simulink library "half_bridge_three_level_ttype_mos_simple_2th"  (R2026a)
settings: Solver=VariableStepAuto
libraries: fl_lib x64, nesl_utility x40, mos_simple_2th_lib x4
(part 1 of 2)
settings Model: Creator=pwr-control  LastModifiedBy=pwr-control

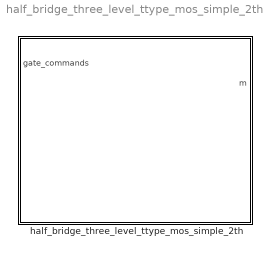
== system half_bridge_three_level_ttype_mos_simple_2th ==
  half_bridge_three_level_ttype_mos_simple_2th : Subsystem  mask(half_bridge_three_level_ttype_mos_simple_2th){rds_on_m=2.6, alpha_R_m=0, Tj_ref_m=125, Roff_m=1e7, v_gamma_m=4.5, rd_on_m=0.185, two_die_m=0, G_th_m=0.5, Eon_m=24, Eoff_m=8, Err_m=1.1, Ic_ref_m=450, Vdc_ref_m=600, ki_m=1, kv_m=1, Vth_off_m=50, Vth_on_m=25, V_sm_m=10, time_constant_edge_m=0.1, tau_v_m=10, time_constant_ploss_m=200, i_eps_m=1e-3, Csnubber_m=12e-12, Rsnubber_m=2200, rth_switch_JH_m=0.116, rth_switch_HA_m=0.05, rth_diode_JH_m=0.116, rth_diode_HA_m=0.05, JunctionTermalMass_m=0.2, Tambient_m=40, mass_heatsink_m=1, specific_heat_m=900}
      mask prompts: rds_on_m "On-state resistance at Tj_ref [mOhm]"; alpha_R_m "Rds_on temperature coefficient, 0 disables it [1/K]"; Tj_ref_m "Reference junction temperature of Rds_on [degC]"; Roff_m "Off-state resistance [Ohm]"; v_gamma_m "Diode knee voltage [V]"; rd_on_m "Diode differential resistance [mOhm]"; two_die_m "Diode die: 1 = separate die (losses to Hd), 0 = body diode (losses to Ht)"; G_th_m "Gate threshold: on when the gate command is above G_th"; Eon_m "Turn-on energy at Ic_ref, Vdc_ref [mJ]"; Eoff_m "Turn-off energy at Ic_ref, Vdc_ref [mJ]"; Err_m "Diode recovery energy at Ic_ref, Vdc_ref [mJ]"; Ic_ref_m "Reference current of the energies [A]"; Vdc_ref_m "Reference voltage of the energies [V]"; ki_m "Current exponent of the energy scaling"; kv_m "Voltage exponent of the energy scaling"; Vth_off_m "Turn-off / recovery detection threshold [V]"; Vth_on_m "Turn-on detection threshold (< Vth_off) [V]"; V_sm_m "Smoothing width of the blocking detector [V]"; time_constant_edge_m "Sample-and-hold time constant (<< dead time) [us]"; tau_v_m "Blocking voltage estimator time constant [us]"; time_constant_ploss_m "Energy-to-power lag time constant (2-5 x Tsw) [us]"; i_eps_m "Current smoothing [A]"; Csnubber_m "RC snubber capacitance [F]"; Rsnubber_m "RC snubber resistance [Ohm]"; rth_switch_JH_m "Thermal resistance junction-heatsink, transistor die [K/W]"; rth_switch_HA_m "Thermal resistance heatsink-ambient, transistor die [K/W]"; rth_diode_JH_m "Thermal resistance junction-heatsink, diode die [K/W]"; rth_diode_HA_m "Thermal resistance heatsink-ambient, diode die [K/W]"; JunctionTermalMass_m "Junction thermal mass of each die [J/K]"; Tambient_m "Ambient temperature [degC]"; mass_heatsink_m "Heatsink mass seen by each die [kg]"; specific_heat_m "Specific heat of the heatsink [J/(K kg)]"
      mask help: Half bridge, three-level T-type, mos_simple_2th devices. MOSFET cells built on mos_simple_2th (library/foundation/semiconductors): resistive bidirectional channel (synchronous rectification), piecewise-linear diode, switching energies scaled from one datasheet point, optional Rds_on temperature coefficient, separate thermal ports for the channel and the diode die (two_die = 0 charges the body diode losses to the transistor die). Each die drives its own junction thermal mass -> Rth JH -> heatsink mass -> Rth HA -> ambient temperature source. The gate command is compared with G_th (works with 0/1 logic and with +15/-10 V). Bus m per device k: mosfet_current, mosfet_voltage, mosfet_ploss, mosfet_JH_temp, mosfet_HA_temp, diode_current, diode_ploss, diode_JH_temp, diode_HA_temp (temperatures are differences in K). Default data: Wolfspeed CAB450M12XM3. Ports: gate_commands (bus from the three-level PWM modulators of masked_models/modulators), m (measurement bus), left dc terminals udc(+) / np / udc(-), right ac terminals u. Device numbering: see half_bridge/README.md.
      mask Help: web('https://github.com/pwr-control/library/blob/dev/library/masked_models/semiconductors_bridges/half_bridge/README.md', '-browser')
      mask DialogControl ParameterGroupVar Prompt: Conduction
      mask DialogControl ParameterGroupVar1 Prompt: Gate
      mask DialogControl ParameterGroupVar2 Prompt: Switching energies
      mask DialogControl ParameterGroupVar3 Prompt: Numerics and snubber
      mask DialogControl ParameterGroupVar4 Prompt: Thermal network
      mask Display:
      | disp(sprintf('half bridge\nT-type 3 levels\nmos_simple_2th'))
      | port_label('input', 1, 'gate_commands')
      | port_label('output', 1, 'm')
      | port_label('LConn', 1, 'udc(+)')
      | port_label('LConn', 2, 'np')
      | port_label('LConn', 3, 'udc(-)')
      | port_label('RConn', 1, 'u')

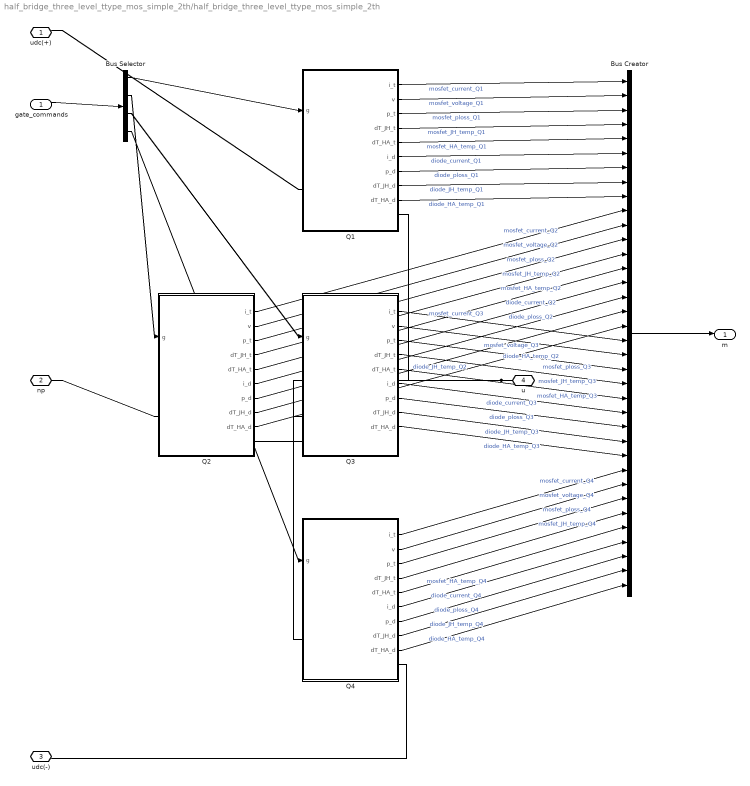
== system half_bridge_three_level_ttype_mos_simple_2th/half_bridge_three_level_ttype_mos_simple_2th ==
  gate_commands : Inport
  Bus Selector : BusSelector  OutputSignals=cmd_gate_Q1,cmd_gate_Q2,cmd_gate_Q3,cmd_gate_Q4
  udc(+) : PMIOPort  Side=Left
  np : PMIOPort  Port=2  Side=Left
  udc(-) : PMIOPort  Port=3  Side=Left
  u : PMIOPort  Port=4  Side=Right
  Bus Creator : BusCreator  Inputs=36
  m : Outport
  Q1 : Subsystem
  Q2 : Subsystem
  Q3 : Subsystem
  Q4 : Subsystem
  wires:
  gate_commands/1 -> Bus Selector/1
  Bus Creator/1 -> m/1
  Bus Selector/1 -> Q1/1(g)
  Q1/1(i_t) -> Bus Creator/1  "mosfet_current_Q1"
  Q1/2(v) -> Bus Creator/2  "mosfet_voltage_Q1"
  Q1/3(p_t) -> Bus Creator/3  "mosfet_ploss_Q1"
  Q1/4(dT_JH_t) -> Bus Creator/4  "mosfet_JH_temp_Q1"
  Q1/5(dT_HA_t) -> Bus Creator/5  "mosfet_HA_temp_Q1"
  Q1/6(i_d) -> Bus Creator/6  "diode_current_Q1"
  Q1/7(p_d) -> Bus Creator/7  "diode_ploss_Q1"
  Q1/8(dT_JH_d) -> Bus Creator/8  "diode_JH_temp_Q1"
  Q1/9(dT_HA_d) -> Bus Creator/9  "diode_HA_temp_Q1"
  Bus Selector/2 -> Q2/1(g)
  Q2/1(i_t) -> Bus Creator/10  "mosfet_current_Q2"
  Q2/2(v) -> Bus Creator/11  "mosfet_voltage_Q2"
  Q2/3(p_t) -> Bus Creator/12  "mosfet_ploss_Q2"
  Q2/4(dT_JH_t) -> Bus Creator/13  "mosfet_JH_temp_Q2"
  Q2/5(dT_HA_t) -> Bus Creator/14  "mosfet_HA_temp_Q2"
  Q2/6(i_d) -> Bus Creator/15  "diode_current_Q2"
  Q2/7(p_d) -> Bus Creator/16  "diode_ploss_Q2"
  Q2/8(dT_JH_d) -> Bus Creator/17  "diode_JH_temp_Q2"
  Q2/9(dT_HA_d) -> Bus Creator/18  "diode_HA_temp_Q2"
  Bus Selector/3 -> Q3/1(g)
  Q3/1(i_t) -> Bus Creator/19  "mosfet_current_Q3"
  Q3/2(v) -> Bus Creator/20  "mosfet_voltage_Q3"
  Q3/3(p_t) -> Bus Creator/21  "mosfet_ploss_Q3"
  Q3/4(dT_JH_t) -> Bus Creator/22  "mosfet_JH_temp_Q3"
  Q3/5(dT_HA_t) -> Bus Creator/23  "mosfet_HA_temp_Q3"
  Q3/6(i_d) -> Bus Creator/24  "diode_current_Q3"
  Q3/7(p_d) -> Bus Creator/25  "diode_ploss_Q3"
  Q3/8(dT_JH_d) -> Bus Creator/26  "diode_JH_temp_Q3"
  Q3/9(dT_HA_d) -> Bus Creator/27  "diode_HA_temp_Q3"
  Bus Selector/4 -> Q4/1(g)
  Q4/1(i_t) -> Bus Creator/28  "mosfet_current_Q4"
  Q4/2(v) -> Bus Creator/29  "mosfet_voltage_Q4"
  Q4/3(p_t) -> Bus Creator/30  "mosfet_ploss_Q4"
  Q4/4(dT_JH_t) -> Bus Creator/31  "mosfet_JH_temp_Q4"
  Q4/5(dT_HA_t) -> Bus Creator/32  "mosfet_HA_temp_Q4"
  Q4/6(i_d) -> Bus Creator/33  "diode_current_Q4"
  Q4/7(p_d) -> Bus Creator/34  "diode_ploss_Q4"
  Q4/8(dT_JH_d) -> Bus Creator/35  "diode_JH_temp_Q4"
  Q4/9(dT_HA_d) -> Bus Creator/36  "diode_HA_temp_Q4"
  connections:
  Q2/RConn1 -- Q3/RConn1
  u/RConn1 -- Q1/RConn1 -- Q4/LConn1 -- Q3/LConn1
  udc(+)/RConn1 -- Q1/LConn1
  udc(-)/RConn1 -- Q4/RConn1
  np/RConn1 -- Q2/LConn1

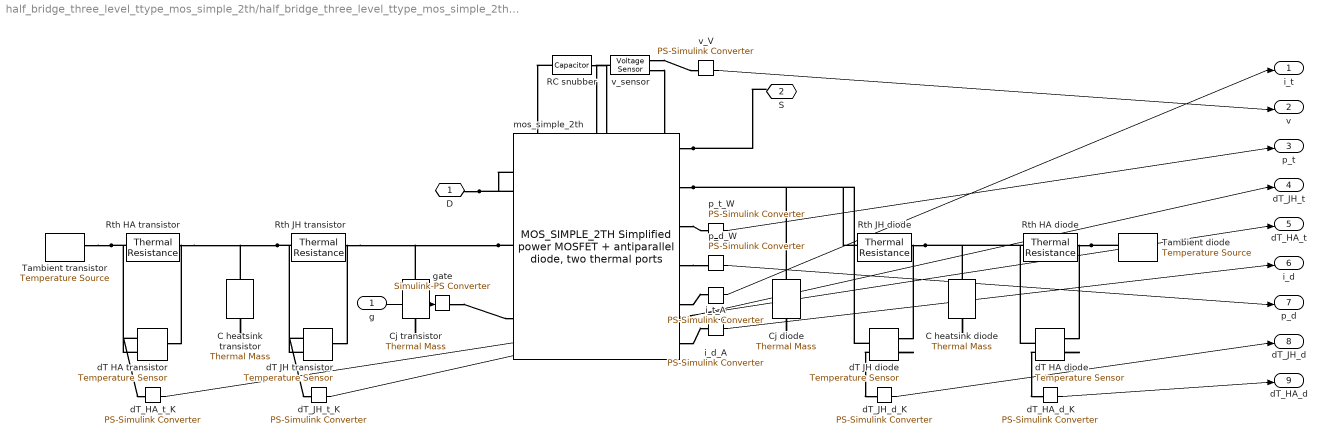
== system half_bridge_three_level_ttype_mos_simple_2th/half_bridge_three_level_ttype_mos_simple_2th/Q1 ==
  g : Inport
  gate : nesl_utility/Simulink-PS Converter  PhysicalDomain=network_engine_domain  SubClassName=ps_input  LeftPortType=input  RightPortType=output  PseudoPeriodic=off  Frequencies=[]  NoiseDistribution=none  NoiseParameters=[]  Unit=1  AffineConversion=off  FilteringAndDerivatives=provide  SimscapeFilterOrder=1  InputFilterTimeConstant=0.001  UdotUserProvided=0
  mos_simple_2th : mos_simple_2th_lib/MOS_SIMPLE_2TH Simplified power MOSFET + antiparallel diode, two thermal ports  Rds_on=rds_on_m mOhm  alpha_R=alpha_R_m 1/K  Tj_ref=Tj_ref_m degC  Roff=Roff_m Ohm  Vf=v_gamma_m V  Rd=rd_on_m mOhm  two_die=two_die_m  G_th=G_th_m  Eon_ref=Eon_m mJ  Eoff_ref=Eoff_m mJ  Err_ref=Err_m mJ  Iref=Ic_ref_m A  Vref=Vdc_ref_m V  ki=ki_m  kv=kv_m  Vth_off=Vth_off_m V  Vth_on=Vth_on_m V  V_sm=V_sm_m V  tau_s=time_constant_edge_m us  tau_v=tau_v_m us  tau_p=time_constant_ploss_m us  i_eps=i_eps_m A  v_eps=1e-3 V  v_specify=off  v_priority=None  v=0 V  v_nominal_specify=off  v_nominal_value=1  v_nominal_unit=V  i_specify=off  i_priority=None  i=0 A  i_nominal_specify=off  i_nominal_value=1  i_nominal_unit=A  ich_specify=off  ich_priority=None  ich=0 A  ich_nominal_specify=off  ich_nominal_value=1  ich_nominal_unit=A  ichp_specify=off  ichp_priority=None  ichp=0 A  ichp_nominal_specify=off  ichp_nominal_value=1  ichp_nominal_unit=A  idio_specify=off  idio_priority=None  idio=0 A  idio_nominal_specify=off  idio_nominal_value=1  idio_nominal_unit=A  vfd_specify=off  vfd_priority=None  vfd=0 V  vfd_nominal_specify=off  vfd_nominal_value=1  vfd_nominal_unit=V  ith_specify=off  ith_priority=None  ith=0 A  ith_nominal_specify=off  ith_nominal_value=1  ith_nominal_unit=A  idh_specify=off  idh_priority=None  idh=0 A  idh_nominal_specify=off  idh_nominal_value=1  idh_nominal_unit=A  vbl_specify=off  vbl_priority=None  vbl=600 V  vbl_nominal_specify=off  vbl_nominal_value=1  vbl_nominal_unit=V  hb_specify=off  hb_priority=None  hb=0  hb_nominal_specify=off  hb_nominal_value=1  hb_nominal_unit=1  Gch_specify=off  Gch_priority=None  Gch=0 S  Gch_nominal_specify=off  Gch_nominal_value=1  Gch_nominal_unit=S  gl_specify=off  gl_priority=None  gl=0  gl_nominal_specify=off  gl_nominal_value=1  gl_nominal_unit=1  Rds_specify=off  Rds_priority=None  Rds=1e-3 Ohm  Rds_nominal_specify=off  Rds_nominal_value=1  Rds_nominal_unit=Ohm  xr_specify=off  xr_priority=None  xr=1  xr_nominal_specify=off  xr_nominal_value=1  xr_nominal_unit=1  Eot_specify=off  Eot_priority=None  Eot=0 J  Eot_nominal_specify=off  Eot_nominal_value=1  Eot_nominal_unit=J  Eod_specify=off  Eod_priority=None  Eod=0 J  Eod_nominal_specify=off  Eod_nominal_value=1  Eod_nominal_unit=J  Pswt_specify=off  Pswt_priority=None  Pswt=0 W  Pswt_nominal_specify=off  Pswt_nominal_value=1  Pswt_nominal_unit=W  Pswd_specify=off  Pswd_priority=None  Pswd=0 W  Pswd_nominal_specify=off  Pswd_nominal_value=1  Pswd_nominal_unit=W  Pct_specify=off  Pct_priority=None  Pct=0 W  Pct_nominal_specify=off  Pct_nominal_value=1  Pct_nominal_unit=W  Pcd_specify=off  Pcd_priority=None  Pcd=0 W  Pcd_nominal_specify=off  Pcd_nominal_value=1  Pcd_nominal_unit=W  Qt_specify=off  Qt_priority=None  Qt=0 W  Qt_nominal_specify=off  Qt_nominal_value=1  Qt_nominal_unit=W  Qd_specify=off  Qd_priority=None  Qd=0 W  Qd_nominal_specify=off  Qd_nominal_value=1  Qd_nominal_unit=W  Eqt_specify=off  Eqt_priority=None  Eqt=0 J  Eqd_specify=off  Eqd_priority=None  Eqd=0 J
  D : PMIOPort  Side=Left
  S : PMIOPort  Port=2  Side=Right
  RC snubber : fl_lib/Electrical/Electrical Elements/Capacitor  c=Csnubber_m F  r=Rsnubber_m Ohm  g=0 1/Ohm  i_specify=off  i_priority=None  i=0 A  i_nominal_specify=off  i_nominal_value=1  i_nominal_unit=A  v_specify=off  v_priority=None  v=0 V  v_nominal_specify=off  v_nominal_value=1  v_nominal_unit=V  vc_specify=off  vc_priority=High  vc=0 V  vc_nominal_specify=off  vc_nominal_value=1  vc_nominal_unit=V
  v_sensor : fl_lib/Electrical/Electrical Sensors/Voltage Sensor
  v_V : nesl_utility/PS-Simulink Converter  PhysicalDomain=network_engine_domain  SubClassName=ps_output  LeftPortType=input  RightPortType=output  PseudoPeriodic=off  Frequencies=[]  VectorFormat=1-D array  Unit=V  AffineConversion=off
  p_t_W : nesl_utility/PS-Simulink Converter  PhysicalDomain=network_engine_domain  SubClassName=ps_output  LeftPortType=input  RightPortType=output  PseudoPeriodic=off  Frequencies=[]  VectorFormat=1-D array  Unit=W  AffineConversion=off
  p_d_W : nesl_utility/PS-Simulink Converter  PhysicalDomain=network_engine_domain  SubClassName=ps_output  LeftPortType=input  RightPortType=output  PseudoPeriodic=off  Frequencies=[]  VectorFormat=1-D array  Unit=W  AffineConversion=off
  i_t_A : nesl_utility/PS-Simulink Converter  PhysicalDomain=network_engine_domain  SubClassName=ps_output  LeftPortType=input  RightPortType=output  PseudoPeriodic=off  Frequencies=[]  VectorFormat=1-D array  Unit=A  AffineConversion=off
  i_d_A : nesl_utility/PS-Simulink Converter  PhysicalDomain=network_engine_domain  SubClassName=ps_output  LeftPortType=input  RightPortType=output  PseudoPeriodic=off  Frequencies=[]  VectorFormat=1-D array  Unit=A  AffineConversion=off
  Cj transistor : fl_lib/Thermal/Thermal Elements/Thermal Mass  mass_type=foundation.enum.constant_variable.constant  mass=JunctionTermalMass_m/specific_heat_m kg  sp_heat=specific_heat_m J/(K*kg)  mass_min=1e-6 kg  num_ports=foundation.enum.numPorts2.one  m_specify=off  m_priority=High  m=1 kg  m_nominal_specify=off  m_nominal_value=1  m_nominal_unit=kg  T_specify=on  T_priority=High  T=Tambient_m degC  T_nominal_specify=off  T_nominal_value=1  T_nominal_unit=K  Q_specify=off  Q_priority=High  Q=0 W  Q_nominal_specify=off  Q_nominal_value=1  Q_nominal_unit=W
  Rth JH transistor : fl_lib/Thermal/Thermal Elements/Thermal Resistance  resistance=rth_switch_JH_m K/W  T_specify=off  T_priority=High  T=0 deltadegC  T_nominal_specify=off  T_nominal_value=1  T_nominal_unit=K  Q_specify=off  Q_priority=None  Q=0 W  Q_nominal_specify=off  Q_nominal_value=1  Q_nominal_unit=W
  C heatsink transistor : fl_lib/Thermal/Thermal Elements/Thermal Mass  mass_type=foundation.enum.constant_variable.constant  mass=mass_heatsink_m kg  sp_heat=specific_heat_m J/(K*kg)  mass_min=1e-6 kg  num_ports=foundation.enum.numPorts2.one  m_specify=off  m_priority=High  m=1 kg  m_nominal_specify=off  m_nominal_value=1  m_nominal_unit=kg  T_specify=on  T_priority=High  T=Tambient_m degC  T_nominal_specify=off  T_nominal_value=1  T_nominal_unit=K  Q_specify=off  Q_priority=High  Q=0 W  Q_nominal_specify=off  Q_nominal_value=1  Q_nominal_unit=W
  Rth HA transistor : fl_lib/Thermal/Thermal Elements/Thermal Resistance  resistance=rth_switch_HA_m K/W  T_specify=off  T_priority=High  T=0 deltadegC  T_nominal_specify=off  T_nominal_value=1  T_nominal_unit=K  Q_specify=off  Q_priority=None  Q=0 W  Q_nominal_specify=off  Q_nominal_value=1  Q_nominal_unit=W
  Tambient transistor : fl_lib/Thermal/Thermal Sources/Temperature Source  temperature=Tambient_m degC
  dT JH transistor : fl_lib/Thermal/Thermal Sensors/Temperature Sensor  temperature_measure=foundation.enum.MeasurementReference.difference
  dT HA transistor : fl_lib/Thermal/Thermal Sensors/Temperature Sensor  temperature_measure=foundation.enum.MeasurementReference.difference
  dT_JH_t_K : nesl_utility/PS-Simulink Converter  PhysicalDomain=network_engine_domain  SubClassName=ps_output  LeftPortType=input  RightPortType=output  PseudoPeriodic=off  Frequencies=[]  VectorFormat=1-D array  Unit=K  AffineConversion=off
  dT_HA_t_K : nesl_utility/PS-Simulink Converter  PhysicalDomain=network_engine_domain  SubClassName=ps_output  LeftPortType=input  RightPortType=output  PseudoPeriodic=off  Frequencies=[]  VectorFormat=1-D array  Unit=K  AffineConversion=off
  Cj diode : fl_lib/Thermal/Thermal Elements/Thermal Mass  mass_type=foundation.enum.constant_variable.constant  mass=JunctionTermalMass_m/specific_heat_m kg  sp_heat=specific_heat_m J/(K*kg)  mass_min=1e-6 kg  num_ports=foundation.enum.numPorts2.one  m_specify=off  m_priority=High  m=1 kg  m_nominal_specify=off  m_nominal_value=1  m_nominal_unit=kg  T_specify=on  T_priority=High  T=Tambient_m degC  T_nominal_specify=off  T_nominal_value=1  T_nominal_unit=K  Q_specify=off  Q_priority=High  Q=0 W  Q_nominal_specify=off  Q_nominal_value=1  Q_nominal_unit=W
  Rth JH diode : fl_lib/Thermal/Thermal Elements/Thermal Resistance  resistance=rth_diode_JH_m K/W  T_specify=off  T_priority=High  T=0 deltadegC  T_nominal_specify=off  T_nominal_value=1  T_nominal_unit=K  Q_specify=off  Q_priority=None  Q=0 W  Q_nominal_specify=off  Q_nominal_value=1  Q_nominal_unit=W
  C heatsink diode : fl_lib/Thermal/Thermal Elements/Thermal Mass  mass_type=foundation.enum.constant_variable.constant  mass=mass_heatsink_m kg  sp_heat=specific_heat_m J/(K*kg)  mass_min=1e-6 kg  num_ports=foundation.enum.numPorts2.one  m_specify=off  m_priority=High  m=1 kg  m_nominal_specify=off  m_nominal_value=1  m_nominal_unit=kg  T_specify=on  T_priority=High  T=Tambient_m degC  T_nominal_specify=off  T_nominal_value=1  T_nominal_unit=K  Q_specify=off  Q_priority=High  Q=0 W  Q_nominal_specify=off  Q_nominal_value=1  Q_nominal_unit=W
  Rth HA diode : fl_lib/Thermal/Thermal Elements/Thermal Resistance  resistance=rth_diode_HA_m K/W  T_specify=off  T_priority=High  T=0 deltadegC  T_nominal_specify=off  T_nominal_value=1  T_nominal_unit=K  Q_specify=off  Q_priority=None  Q=0 W  Q_nominal_specify=off  Q_nominal_value=1  Q_nominal_unit=W
  Tambient diode : fl_lib/Thermal/Thermal Sources/Temperature Source  temperature=Tambient_m degC
  dT JH diode : fl_lib/Thermal/Thermal Sensors/Temperature Sensor  temperature_measure=foundation.enum.MeasurementReference.difference
  dT HA diode : fl_lib/Thermal/Thermal Sensors/Temperature Sensor  temperature_measure=foundation.enum.MeasurementReference.difference
  dT_JH_d_K : nesl_utility/PS-Simulink Converter  PhysicalDomain=network_engine_domain  SubClassName=ps_output  LeftPortType=input  RightPortType=output  PseudoPeriodic=off  Frequencies=[]  VectorFormat=1-D array  Unit=K  AffineConversion=off
  dT_HA_d_K : nesl_utility/PS-Simulink Converter  PhysicalDomain=network_engine_domain  SubClassName=ps_output  LeftPortType=input  RightPortType=output  PseudoPeriodic=off  Frequencies=[]  VectorFormat=1-D array  Unit=K  AffineConversion=off
  i_t : Outport
  v : Outport  Port=2
  p_t : Outport  Port=3
  dT_JH_t : Outport  Port=4
  dT_HA_t : Outport  Port=5
  i_d : Outport  Port=6
  p_d : Outport  Port=7
  dT_JH_d : Outport  Port=8
  dT_HA_d : Outport  Port=9
  wires:
  i_t_A/1 -> i_t/1
  v_V/1 -> v/1
  p_t_W/1 -> p_t/1
  dT_JH_t_K/1 -> dT_JH_t/1
  dT_HA_t_K/1 -> dT_HA_t/1
  i_d_A/1 -> i_d/1
  p_d_W/1 -> p_d/1
  dT_JH_d_K/1 -> dT_JH_d/1
  dT_HA_d_K/1 -> dT_HA_d/1
  g/1 -> gate/1
  connections:
  Rth JH transistor/RConn1 -- C heatsink transistor/LConn1 -- Rth HA transistor/LConn1 -- dT JH transistor/RConn1 -- dT HA transistor/LConn1
  Rth HA transistor/RConn1 -- Tambient transistor/LConn1 -- dT HA transistor/RConn1
  dT JH transistor/RConn2 -- dT_JH_t_K/LConn1
  dT HA transistor/RConn2 -- dT_HA_t_K/LConn1
  Rth JH diode/RConn1 -- C heatsink diode/LConn1 -- Rth HA diode/LConn1 -- dT JH diode/RConn1 -- dT HA diode/LConn1
  Rth HA diode/RConn1 -- Tambient diode/LConn1 -- dT HA diode/RConn1
  dT JH diode/RConn2 -- dT_JH_d_K/LConn1
  dT HA diode/RConn2 -- dT_HA_d_K/LConn1
  gate/RConn1 -- mos_simple_2th/LConn3
  D/RConn1 -- mos_simple_2th/LConn1 -- RC snubber/LConn1 -- v_sensor/LConn1
  mos_simple_2th/RConn1 -- S/RConn1 -- RC snubber/RConn1 -- v_sensor/RConn2
  v_sensor/RConn1 -- v_V/LConn1
  mos_simple_2th/RConn3 -- p_t_W/LConn1
  mos_simple_2th/RConn4 -- p_d_W/LConn1
  mos_simple_2th/RConn5 -- i_t_A/LConn1
  mos_simple_2th/RConn6 -- i_d_A/LConn1
  mos_simple_2th/LConn2 -- Cj transistor/LConn1 -- Rth JH transistor/LConn1 -- dT JH transistor/LConn1
  mos_simple_2th/RConn2 -- Cj diode/LConn1 -- Rth JH diode/LConn1 -- dT JH diode/LConn1

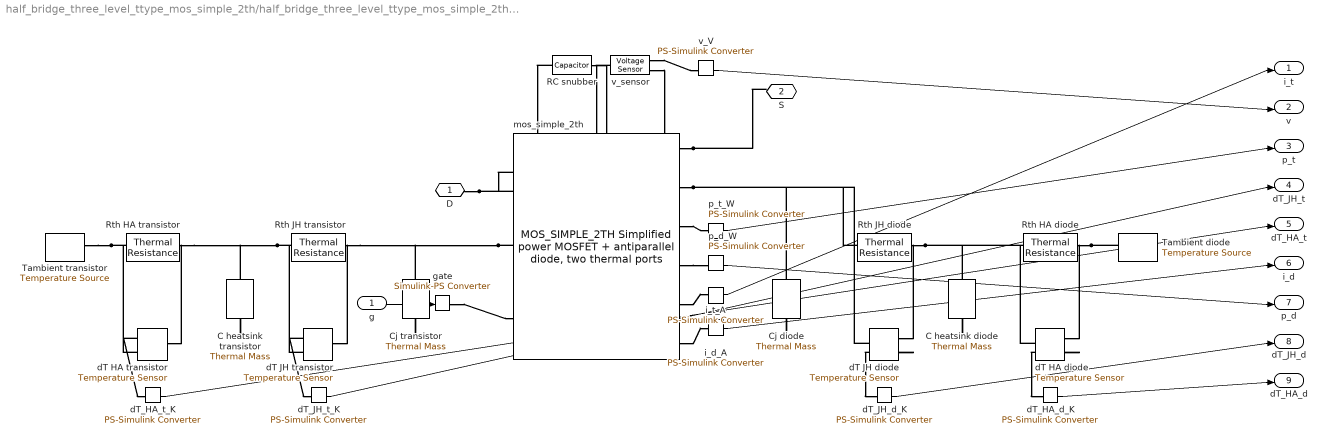
== system half_bridge_three_level_ttype_mos_simple_2th/half_bridge_three_level_ttype_mos_simple_2th/Q2 ==
  g : Inport
  gate : nesl_utility/Simulink-PS Converter  PhysicalDomain=network_engine_domain  SubClassName=ps_input  LeftPortType=input  RightPortType=output  PseudoPeriodic=off  Frequencies=[]  NoiseDistribution=none  NoiseParameters=[]  Unit=1  AffineConversion=off  FilteringAndDerivatives=provide  SimscapeFilterOrder=1  InputFilterTimeConstant=0.001  UdotUserProvided=0
  mos_simple_2th : mos_simple_2th_lib/MOS_SIMPLE_2TH Simplified power MOSFET + antiparallel diode, two thermal ports  Rds_on=rds_on_m mOhm  alpha_R=alpha_R_m 1/K  Tj_ref=Tj_ref_m degC  Roff=Roff_m Ohm  Vf=v_gamma_m V  Rd=rd_on_m mOhm  two_die=two_die_m  G_th=G_th_m  Eon_ref=Eon_m mJ  Eoff_ref=Eoff_m mJ  Err_ref=Err_m mJ  Iref=Ic_ref_m A  Vref=Vdc_ref_m V  ki=ki_m  kv=kv_m  Vth_off=Vth_off_m V  Vth_on=Vth_on_m V  V_sm=V_sm_m V  tau_s=time_constant_edge_m us  tau_v=tau_v_m us  tau_p=time_constant_ploss_m us  i_eps=i_eps_m A  v_eps=1e-3 V  v_specify=off  v_priority=None  v=0 V  v_nominal_specify=off  v_nominal_value=1  v_nominal_unit=V  i_specify=off  i_priority=None  i=0 A  i_nominal_specify=off  i_nominal_value=1  i_nominal_unit=A  ich_specify=off  ich_priority=None  ich=0 A  ich_nominal_specify=off  ich_nominal_value=1  ich_nominal_unit=A  ichp_specify=off  ichp_priority=None  ichp=0 A  ichp_nominal_specify=off  ichp_nominal_value=1  ichp_nominal_unit=A  idio_specify=off  idio_priority=None  idio=0 A  idio_nominal_specify=off  idio_nominal_value=1  idio_nominal_unit=A  vfd_specify=off  vfd_priority=None  vfd=0 V  vfd_nominal_specify=off  vfd_nominal_value=1  vfd_nominal_unit=V  ith_specify=off  ith_priority=None  ith=0 A  ith_nominal_specify=off  ith_nominal_value=1  ith_nominal_unit=A  idh_specify=off  idh_priority=None  idh=0 A  idh_nominal_specify=off  idh_nominal_value=1  idh_nominal_unit=A  vbl_specify=off  vbl_priority=None  vbl=600 V  vbl_nominal_specify=off  vbl_nominal_value=1  vbl_nominal_unit=V  hb_specify=off  hb_priority=None  hb=0  hb_nominal_specify=off  hb_nominal_value=1  hb_nominal_unit=1  Gch_specify=off  Gch_priority=None  Gch=0 S  Gch_nominal_specify=off  Gch_nominal_value=1  Gch_nominal_unit=S  gl_specify=off  gl_priority=None  gl=0  gl_nominal_specify=off  gl_nominal_value=1  gl_nominal_unit=1  Rds_specify=off  Rds_priority=None  Rds=1e-3 Ohm  Rds_nominal_specify=off  Rds_nominal_value=1  Rds_nominal_unit=Ohm  xr_specify=off  xr_priority=None  xr=1  xr_nominal_specify=off  xr_nominal_value=1  xr_nominal_unit=1  Eot_specify=off  Eot_priority=None  Eot=0 J  Eot_nominal_specify=off  Eot_nominal_value=1  Eot_nominal_unit=J  Eod_specify=off  Eod_priority=None  Eod=0 J  Eod_nominal_specify=off  Eod_nominal_value=1  Eod_nominal_unit=J  Pswt_specify=off  Pswt_priority=None  Pswt=0 W  Pswt_nominal_specify=off  Pswt_nominal_value=1  Pswt_nominal_unit=W  Pswd_specify=off  Pswd_priority=None  Pswd=0 W  Pswd_nominal_specify=off  Pswd_nominal_value=1  Pswd_nominal_unit=W  Pct_specify=off  Pct_priority=None  Pct=0 W  Pct_nominal_specify=off  Pct_nominal_value=1  Pct_nominal_unit=W  Pcd_specify=off  Pcd_priority=None  Pcd=0 W  Pcd_nominal_specify=off  Pcd_nominal_value=1  Pcd_nominal_unit=W  Qt_specify=off  Qt_priority=None  Qt=0 W  Qt_nominal_specify=off  Qt_nominal_value=1  Qt_nominal_unit=W  Qd_specify=off  Qd_priority=None  Qd=0 W  Qd_nominal_specify=off  Qd_nominal_value=1  Qd_nominal_unit=W  Eqt_specify=off  Eqt_priority=None  Eqt=0 J  Eqd_specify=off  Eqd_priority=None  Eqd=0 J
  D : PMIOPort  Side=Left
  S : PMIOPort  Port=2  Side=Right
  RC snubber : fl_lib/Electrical/Electrical Elements/Capacitor  c=Csnubber_m F  r=Rsnubber_m Ohm  g=0 1/Ohm  i_specify=off  i_priority=None  i=0 A  i_nominal_specify=off  i_nominal_value=1  i_nominal_unit=A  v_specify=off  v_priority=None  v=0 V  v_nominal_specify=off  v_nominal_value=1  v_nominal_unit=V  vc_specify=off  vc_priority=High  vc=0 V  vc_nominal_specify=off  vc_nominal_value=1  vc_nominal_unit=V
  v_sensor : fl_lib/Electrical/Electrical Sensors/Voltage Sensor
  v_V : nesl_utility/PS-Simulink Converter  PhysicalDomain=network_engine_domain  SubClassName=ps_output  LeftPortType=input  RightPortType=output  PseudoPeriodic=off  Frequencies=[]  VectorFormat=1-D array  Unit=V  AffineConversion=off
  p_t_W : nesl_utility/PS-Simulink Converter  PhysicalDomain=network_engine_domain  SubClassName=ps_output  LeftPortType=input  RightPortType=output  PseudoPeriodic=off  Frequencies=[]  VectorFormat=1-D array  Unit=W  AffineConversion=off
  p_d_W : nesl_utility/PS-Simulink Converter  PhysicalDomain=network_engine_domain  SubClassName=ps_output  LeftPortType=input  RightPortType=output  PseudoPeriodic=off  Frequencies=[]  VectorFormat=1-D array  Unit=W  AffineConversion=off
  i_t_A : nesl_utility/PS-Simulink Converter  PhysicalDomain=network_engine_domain  SubClassName=ps_output  LeftPortType=input  RightPortType=output  PseudoPeriodic=off  Frequencies=[]  VectorFormat=1-D array  Unit=A  AffineConversion=off
  i_d_A : nesl_utility/PS-Simulink Converter  PhysicalDomain=network_engine_domain  SubClassName=ps_output  LeftPortType=input  RightPortType=output  PseudoPeriodic=off  Frequencies=[]  VectorFormat=1-D array  Unit=A  AffineConversion=off
  Cj transistor : fl_lib/Thermal/Thermal Elements/Thermal Mass  mass_type=foundation.enum.constant_variable.constant  mass=JunctionTermalMass_m/specific_heat_m kg  sp_heat=specific_heat_m J/(K*kg)  mass_min=1e-6 kg  num_ports=foundation.enum.numPorts2.one  m_specify=off  m_priority=High  m=1 kg  m_nominal_specify=off  m_nominal_value=1  m_nominal_unit=kg  T_specify=on  T_priority=High  T=Tambient_m degC  T_nominal_specify=off  T_nominal_value=1  T_nominal_unit=K  Q_specify=off  Q_priority=High  Q=0 W  Q_nominal_specify=off  Q_nominal_value=1  Q_nominal_unit=W
  Rth JH transistor : fl_lib/Thermal/Thermal Elements/Thermal Resistance  resistance=rth_switch_JH_m K/W  T_specify=off  T_priority=High  T=0 deltadegC  T_nominal_specify=off  T_nominal_value=1  T_nominal_unit=K  Q_specify=off  Q_priority=None  Q=0 W  Q_nominal_specify=off  Q_nominal_value=1  Q_nominal_unit=W
  C heatsink transistor : fl_lib/Thermal/Thermal Elements/Thermal Mass  mass_type=foundation.enum.constant_variable.constant  mass=mass_heatsink_m kg  sp_heat=specific_heat_m J/(K*kg)  mass_min=1e-6 kg  num_ports=foundation.enum.numPorts2.one  m_specify=off  m_priority=High  m=1 kg  m_nominal_specify=off  m_nominal_value=1  m_nominal_unit=kg  T_specify=on  T_priority=High  T=Tambient_m degC  T_nominal_specify=off  T_nominal_value=1  T_nominal_unit=K  Q_specify=off  Q_priority=High  Q=0 W  Q_nominal_specify=off  Q_nominal_value=1  Q_nominal_unit=W
  Rth HA transistor : fl_lib/Thermal/Thermal Elements/Thermal Resistance  resistance=rth_switch_HA_m K/W  T_specify=off  T_priority=High  T=0 deltadegC  T_nominal_specify=off  T_nominal_value=1  T_nominal_unit=K  Q_specify=off  Q_priority=None  Q=0 W  Q_nominal_specify=off  Q_nominal_value=1  Q_nominal_unit=W
  Tambient transistor : fl_lib/Thermal/Thermal Sources/Temperature Source  temperature=Tambient_m degC
  dT JH transistor : fl_lib/Thermal/Thermal Sensors/Temperature Sensor  temperature_measure=foundation.enum.MeasurementReference.difference
  dT HA transistor : fl_lib/Thermal/Thermal Sensors/Temperature Sensor  temperature_measure=foundation.enum.MeasurementReference.difference
  dT_JH_t_K : nesl_utility/PS-Simulink Converter  PhysicalDomain=network_engine_domain  SubClassName=ps_output  LeftPortType=input  RightPortType=output  PseudoPeriodic=off  Frequencies=[]  VectorFormat=1-D array  Unit=K  AffineConversion=off
  dT_HA_t_K : nesl_utility/PS-Simulink Converter  PhysicalDomain=network_engine_domain  SubClassName=ps_output  LeftPortType=input  RightPortType=output  PseudoPeriodic=off  Frequencies=[]  VectorFormat=1-D array  Unit=K  AffineConversion=off
  Cj diode : fl_lib/Thermal/Thermal Elements/Thermal Mass  mass_type=foundation.enum.constant_variable.constant  mass=JunctionTermalMass_m/specific_heat_m kg  sp_heat=specific_heat_m J/(K*kg)  mass_min=1e-6 kg  num_ports=foundation.enum.numPorts2.one  m_specify=off  m_priority=High  m=1 kg  m_nominal_specify=off  m_nominal_value=1  m_nominal_unit=kg  T_specify=on  T_priority=High  T=Tambient_m degC  T_nominal_specify=off  T_nominal_value=1  T_nominal_unit=K  Q_specify=off  Q_priority=High  Q=0 W  Q_nominal_specify=off  Q_nominal_value=1  Q_nominal_unit=W
  Rth JH diode : fl_lib/Thermal/Thermal Elements/Thermal Resistance  resistance=rth_diode_JH_m K/W  T_specify=off  T_priority=High  T=0 deltadegC  T_nominal_specify=off  T_nominal_value=1  T_nominal_unit=K  Q_specify=off  Q_priority=None  Q=0 W  Q_nominal_specify=off  Q_nominal_value=1  Q_nominal_unit=W
  C heatsink diode : fl_lib/Thermal/Thermal Elements/Thermal Mass  mass_type=foundation.enum.constant_variable.constant  mass=mass_heatsink_m kg  sp_heat=specific_heat_m J/(K*kg)  mass_min=1e-6 kg  num_ports=foundation.enum.numPorts2.one  m_specify=off  m_priority=High  m=1 kg  m_nominal_specify=off  m_nominal_value=1  m_nominal_unit=kg  T_specify=on  T_priority=High  T=Tambient_m degC  T_nominal_specify=off  T_nominal_value=1  T_nominal_unit=K  Q_specify=off  Q_priority=High  Q=0 W  Q_nominal_specify=off  Q_nominal_value=1  Q_nominal_unit=W
  Rth HA diode : fl_lib/Thermal/Thermal Elements/Thermal Resistance  resistance=rth_diode_HA_m K/W  T_specify=off  T_priority=High  T=0 deltadegC  T_nominal_specify=off  T_nominal_value=1  T_nominal_unit=K  Q_specify=off  Q_priority=None  Q=0 W  Q_nominal_specify=off  Q_nominal_value=1  Q_nominal_unit=W
  Tambient diode : fl_lib/Thermal/Thermal Sources/Temperature Source  temperature=Tambient_m degC
  dT JH diode : fl_lib/Thermal/Thermal Sensors/Temperature Sensor  temperature_measure=foundation.enum.MeasurementReference.difference
  dT HA diode : fl_lib/Thermal/Thermal Sensors/Temperature Sensor  temperature_measure=foundation.enum.MeasurementReference.difference
  dT_JH_d_K : nesl_utility/PS-Simulink Converter  PhysicalDomain=network_engine_domain  SubClassName=ps_output  LeftPortType=input  RightPortType=output  PseudoPeriodic=off  Frequencies=[]  VectorFormat=1-D array  Unit=K  AffineConversion=off
  dT_HA_d_K : nesl_utility/PS-Simulink Converter  PhysicalDomain=network_engine_domain  SubClassName=ps_output  LeftPortType=input  RightPortType=output  PseudoPeriodic=off  Frequencies=[]  VectorFormat=1-D array  Unit=K  AffineConversion=off
  i_t : Outport
  v : Outport  Port=2
  p_t : Outport  Port=3
  dT_JH_t : Outport  Port=4
  dT_HA_t : Outport  Port=5
  i_d : Outport  Port=6
  p_d : Outport  Port=7
  dT_JH_d : Outport  Port=8
  dT_HA_d : Outport  Port=9
  wires:
  i_t_A/1 -> i_t/1
  v_V/1 -> v/1
  p_t_W/1 -> p_t/1
  dT_JH_t_K/1 -> dT_JH_t/1
  dT_HA_t_K/1 -> dT_HA_t/1
  i_d_A/1 -> i_d/1
  p_d_W/1 -> p_d/1
  dT_JH_d_K/1 -> dT_JH_d/1
  dT_HA_d_K/1 -> dT_HA_d/1
  g/1 -> gate/1
  connections:
  Rth JH transistor/RConn1 -- C heatsink transistor/LConn1 -- Rth HA transistor/LConn1 -- dT JH transistor/RConn1 -- dT HA transistor/LConn1
  Rth HA transistor/RConn1 -- Tambient transistor/LConn1 -- dT HA transistor/RConn1
  dT JH transistor/RConn2 -- dT_JH_t_K/LConn1
  dT HA transistor/RConn2 -- dT_HA_t_K/LConn1
  Rth JH diode/RConn1 -- C heatsink diode/LConn1 -- Rth HA diode/LConn1 -- dT JH diode/RConn1 -- dT HA diode/LConn1
  Rth HA diode/RConn1 -- Tambient diode/LConn1 -- dT HA diode/RConn1
  dT JH diode/RConn2 -- dT_JH_d_K/LConn1
  dT HA diode/RConn2 -- dT_HA_d_K/LConn1
  gate/RConn1 -- mos_simple_2th/LConn3
  D/RConn1 -- mos_simple_2th/LConn1 -- RC snubber/LConn1 -- v_sensor/LConn1
  mos_simple_2th/RConn1 -- S/RConn1 -- RC snubber/RConn1 -- v_sensor/RConn2
  v_sensor/RConn1 -- v_V/LConn1
  mos_simple_2th/RConn3 -- p_t_W/LConn1
  mos_simple_2th/RConn4 -- p_d_W/LConn1
  mos_simple_2th/RConn5 -- i_t_A/LConn1
  mos_simple_2th/RConn6 -- i_d_A/LConn1
  mos_simple_2th/LConn2 -- Cj transistor/LConn1 -- Rth JH transistor/LConn1 -- dT JH transistor/LConn1
  mos_simple_2th/RConn2 -- Cj diode/LConn1 -- Rth JH diode/LConn1 -- dT JH diode/LConn1

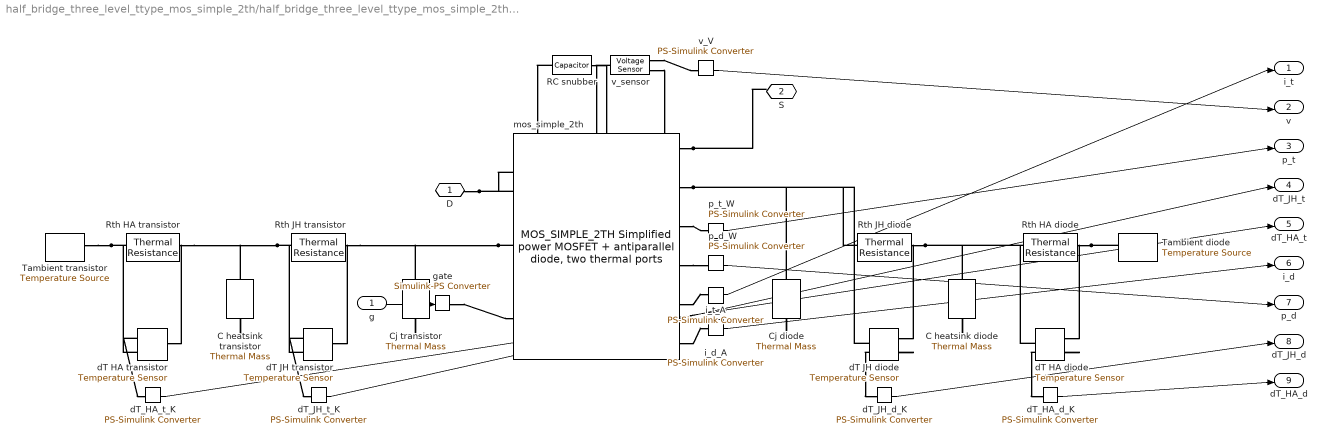
== system half_bridge_three_level_ttype_mos_simple_2th/half_bridge_three_level_ttype_mos_simple_2th/Q3 ==
  g : Inport
  gate : nesl_utility/Simulink-PS Converter  PhysicalDomain=network_engine_domain  SubClassName=ps_input  LeftPortType=input  RightPortType=output  PseudoPeriodic=off  Frequencies=[]  NoiseDistribution=none  NoiseParameters=[]  Unit=1  AffineConversion=off  FilteringAndDerivatives=provide  SimscapeFilterOrder=1  InputFilterTimeConstant=0.001  UdotUserProvided=0
  mos_simple_2th : mos_simple_2th_lib/MOS_SIMPLE_2TH Simplified power MOSFET + antiparallel diode, two thermal ports  Rds_on=rds_on_m mOhm  alpha_R=alpha_R_m 1/K  Tj_ref=Tj_ref_m degC  Roff=Roff_m Ohm  Vf=v_gamma_m V  Rd=rd_on_m mOhm  two_die=two_die_m  G_th=G_th_m  Eon_ref=Eon_m mJ  Eoff_ref=Eoff_m mJ  Err_ref=Err_m mJ  Iref=Ic_ref_m A  Vref=Vdc_ref_m V  ki=ki_m  kv=kv_m  Vth_off=Vth_off_m V  Vth_on=Vth_on_m V  V_sm=V_sm_m V  tau_s=time_constant_edge_m us  tau_v=tau_v_m us  tau_p=time_constant_ploss_m us  i_eps=i_eps_m A  v_eps=1e-3 V  v_specify=off  v_priority=None  v=0 V  v_nominal_specify=off  v_nominal_value=1  v_nominal_unit=V  i_specify=off  i_priority=None  i=0 A  i_nominal_specify=off  i_nominal_value=1  i_nominal_unit=A  ich_specify=off  ich_priority=None  ich=0 A  ich_nominal_specify=off  ich_nominal_value=1  ich_nominal_unit=A  ichp_specify=off  ichp_priority=None  ichp=0 A  ichp_nominal_specify=off  ichp_nominal_value=1  ichp_nominal_unit=A  idio_specify=off  idio_priority=None  idio=0 A  idio_nominal_specify=off  idio_nominal_value=1  idio_nominal_unit=A  vfd_specify=off  vfd_priority=None  vfd=0 V  vfd_nominal_specify=off  vfd_nominal_value=1  vfd_nominal_unit=V  ith_specify=off  ith_priority=None  ith=0 A  ith_nominal_specify=off  ith_nominal_value=1  ith_nominal_unit=A  idh_specify=off  idh_priority=None  idh=0 A  idh_nominal_specify=off  idh_nominal_value=1  idh_nominal_unit=A  vbl_specify=off  vbl_priority=None  vbl=600 V  vbl_nominal_specify=off  vbl_nominal_value=1  vbl_nominal_unit=V  hb_specify=off  hb_priority=None  hb=0  hb_nominal_specify=off  hb_nominal_value=1  hb_nominal_unit=1  Gch_specify=off  Gch_priority=None  Gch=0 S  Gch_nominal_specify=off  Gch_nominal_value=1  Gch_nominal_unit=S  gl_specify=off  gl_priority=None  gl=0  gl_nominal_specify=off  gl_nominal_value=1  gl_nominal_unit=1  Rds_specify=off  Rds_priority=None  Rds=1e-3 Ohm  Rds_nominal_specify=off  Rds_nominal_value=1  Rds_nominal_unit=Ohm  xr_specify=off  xr_priority=None  xr=1  xr_nominal_specify=off  xr_nominal_value=1  xr_nominal_unit=1  Eot_specify=off  Eot_priority=None  Eot=0 J  Eot_nominal_specify=off  Eot_nominal_value=1  Eot_nominal_unit=J  Eod_specify=off  Eod_priority=None  Eod=0 J  Eod_nominal_specify=off  Eod_nominal_value=1  Eod_nominal_unit=J  Pswt_specify=off  Pswt_priority=None  Pswt=0 W  Pswt_nominal_specify=off  Pswt_nominal_value=1  Pswt_nominal_unit=W  Pswd_specify=off  Pswd_priority=None  Pswd=0 W  Pswd_nominal_specify=off  Pswd_nominal_value=1  Pswd_nominal_unit=W  Pct_specify=off  Pct_priority=None  Pct=0 W  Pct_nominal_specify=off  Pct_nominal_value=1  Pct_nominal_unit=W  Pcd_specify=off  Pcd_priority=None  Pcd=0 W  Pcd_nominal_specify=off  Pcd_nominal_value=1  Pcd_nominal_unit=W  Qt_specify=off  Qt_priority=None  Qt=0 W  Qt_nominal_specify=off  Qt_nominal_value=1  Qt_nominal_unit=W  Qd_specify=off  Qd_priority=None  Qd=0 W  Qd_nominal_specify=off  Qd_nominal_value=1  Qd_nominal_unit=W  Eqt_specify=off  Eqt_priority=None  Eqt=0 J  Eqd_specify=off  Eqd_priority=None  Eqd=0 J
  D : PMIOPort  Side=Left
  S : PMIOPort  Port=2  Side=Right
  RC snubber : fl_lib/Electrical/Electrical Elements/Capacitor  c=Csnubber_m F  r=Rsnubber_m Ohm  g=0 1/Ohm  i_specify=off  i_priority=None  i=0 A  i_nominal_specify=off  i_nominal_value=1  i_nominal_unit=A  v_specify=off  v_priority=None  v=0 V  v_nominal_specify=off  v_nominal_value=1  v_nominal_unit=V  vc_specify=off  vc_priority=High  vc=0 V  vc_nominal_specify=off  vc_nominal_value=1  vc_nominal_unit=V
  v_sensor : fl_lib/Electrical/Electrical Sensors/Voltage Sensor
  v_V : nesl_utility/PS-Simulink Converter  PhysicalDomain=network_engine_domain  SubClassName=ps_output  LeftPortType=input  RightPortType=output  PseudoPeriodic=off  Frequencies=[]  VectorFormat=1-D array  Unit=V  AffineConversion=off
  p_t_W : nesl_utility/PS-Simulink Converter  PhysicalDomain=network_engine_domain  SubClassName=ps_output  LeftPortType=input  RightPortType=output  PseudoPeriodic=off  Frequencies=[]  VectorFormat=1-D array  Unit=W  AffineConversion=off
  p_d_W : nesl_utility/PS-Simulink Converter  PhysicalDomain=network_engine_domain  SubClassName=ps_output  LeftPortType=input  RightPortType=output  PseudoPeriodic=off  Frequencies=[]  VectorFormat=1-D array  Unit=W  AffineConversion=off
  i_t_A : nesl_utility/PS-Simulink Converter  PhysicalDomain=network_engine_domain  SubClassName=ps_output  LeftPortType=input  RightPortType=output  PseudoPeriodic=off  Frequencies=[]  VectorFormat=1-D array  Unit=A  AffineConversion=off
  i_d_A : nesl_utility/PS-Simulink Converter  PhysicalDomain=network_engine_domain  SubClassName=ps_output  LeftPortType=input  RightPortType=output  PseudoPeriodic=off  Frequencies=[]  VectorFormat=1-D array  Unit=A  AffineConversion=off
  Cj transistor : fl_lib/Thermal/Thermal Elements/Thermal Mass  mass_type=foundation.enum.constant_variable.constant  mass=JunctionTermalMass_m/specific_heat_m kg  sp_heat=specific_heat_m J/(K*kg)  mass_min=1e-6 kg  num_ports=foundation.enum.numPorts2.one  m_specify=off  m_priority=High  m=1 kg  m_nominal_specify=off  m_nominal_value=1  m_nominal_unit=kg  T_specify=on  T_priority=High  T=Tambient_m degC  T_nominal_specify=off  T_nominal_value=1  T_nominal_unit=K  Q_specify=off  Q_priority=High  Q=0 W  Q_nominal_specify=off  Q_nominal_value=1  Q_nominal_unit=W
  Rth JH transistor : fl_lib/Thermal/Thermal Elements/Thermal Resistance  resistance=rth_switch_JH_m K/W  T_specify=off  T_priority=High  T=0 deltadegC  T_nominal_specify=off  T_nominal_value=1  T_nominal_unit=K  Q_specify=off  Q_priority=None  Q=0 W  Q_nominal_specify=off  Q_nominal_value=1  Q_nominal_unit=W
  C heatsink transistor : fl_lib/Thermal/Thermal Elements/Thermal Mass  mass_type=foundation.enum.constant_variable.constant  mass=mass_heatsink_m kg  sp_heat=specific_heat_m J/(K*kg)  mass_min=1e-6 kg  num_ports=foundation.enum.numPorts2.one  m_specify=off  m_priority=High  m=1 kg  m_nominal_specify=off  m_nominal_value=1  m_nominal_unit=kg  T_specify=on  T_priority=High  T=Tambient_m degC  T_nominal_specify=off  T_nominal_value=1  T_nominal_unit=K  Q_specify=off  Q_priority=High  Q=0 W  Q_nominal_specify=off  Q_nominal_value=1  Q_nominal_unit=W
  Rth HA transistor : fl_lib/Thermal/Thermal Elements/Thermal Resistance  resistance=rth_switch_HA_m K/W  T_specify=off  T_priority=High  T=0 deltadegC  T_nominal_specify=off  T_nominal_value=1  T_nominal_unit=K  Q_specify=off  Q_priority=None  Q=0 W  Q_nominal_specify=off  Q_nominal_value=1  Q_nominal_unit=W
  Tambient transistor : fl_lib/Thermal/Thermal Sources/Temperature Source  temperature=Tambient_m degC
  dT JH transistor : fl_lib/Thermal/Thermal Sensors/Temperature Sensor  temperature_measure=foundation.enum.MeasurementReference.difference
  dT HA transistor : fl_lib/Thermal/Thermal Sensors/Temperature Sensor  temperature_measure=foundation.enum.MeasurementReference.difference
  dT_JH_t_K : nesl_utility/PS-Simulink Converter  PhysicalDomain=network_engine_domain  SubClassName=ps_output  LeftPortType=input  RightPortType=output  PseudoPeriodic=off  Frequencies=[]  VectorFormat=1-D array  Unit=K  AffineConversion=off
  dT_HA_t_K : nesl_utility/PS-Simulink Converter  PhysicalDomain=network_engine_domain  SubClassName=ps_output  LeftPortType=input  RightPortType=output  PseudoPeriodic=off  Frequencies=[]  VectorFormat=1-D array  Unit=K  AffineConversion=off
  Cj diode : fl_lib/Thermal/Thermal Elements/Thermal Mass  mass_type=foundation.enum.constant_variable.constant  mass=JunctionTermalMass_m/specific_heat_m kg  sp_heat=specific_heat_m J/(K*kg)  mass_min=1e-6 kg  num_ports=foundation.enum.numPorts2.one  m_specify=off  m_priority=High  m=1 kg  m_nominal_specify=off  m_nominal_value=1  m_nominal_unit=kg  T_specify=on  T_priority=High  T=Tambient_m degC  T_nominal_specify=off  T_nominal_value=1  T_nominal_unit=K  Q_specify=off  Q_priority=High  Q=0 W  Q_nominal_specify=off  Q_nominal_value=1  Q_nominal_unit=W
  Rth JH diode : fl_lib/Thermal/Thermal Elements/Thermal Resistance  resistance=rth_diode_JH_m K/W  T_specify=off  T_priority=High  T=0 deltadegC  T_nominal_specify=off  T_nominal_value=1  T_nominal_unit=K  Q_specify=off  Q_priority=None  Q=0 W  Q_nominal_specify=off  Q_nominal_value=1  Q_nominal_unit=W
  C heatsink diode : fl_lib/Thermal/Thermal Elements/Thermal Mass  mass_type=foundation.enum.constant_variable.constant  mass=mass_heatsink_m kg  sp_heat=specific_heat_m J/(K*kg)  mass_min=1e-6 kg  num_ports=foundation.enum.numPorts2.one  m_specify=off  m_priority=High  m=1 kg  m_nominal_specify=off  m_nominal_value=1  m_nominal_unit=kg  T_specify=on  T_priority=High  T=Tambient_m degC  T_nominal_specify=off  T_nominal_value=1  T_nominal_unit=K  Q_specify=off  Q_priority=High  Q=0 W  Q_nominal_specify=off  Q_nominal_value=1  Q_nominal_unit=W
  Rth HA diode : fl_lib/Thermal/Thermal Elements/Thermal Resistance  resistance=rth_diode_HA_m K/W  T_specify=off  T_priority=High  T=0 deltadegC  T_nominal_specify=off  T_nominal_value=1  T_nominal_unit=K  Q_specify=off  Q_priority=None  Q=0 W  Q_nominal_specify=off  Q_nominal_value=1  Q_nominal_unit=W
  Tambient diode : fl_lib/Thermal/Thermal Sources/Temperature Source  temperature=Tambient_m degC
  dT JH diode : fl_lib/Thermal/Thermal Sensors/Temperature Sensor  temperature_measure=foundation.enum.MeasurementReference.difference
  dT HA diode : fl_lib/Thermal/Thermal Sensors/Temperature Sensor  temperature_measure=foundation.enum.MeasurementReference.difference
  dT_JH_d_K : nesl_utility/PS-Simulink Converter  PhysicalDomain=network_engine_domain  SubClassName=ps_output  LeftPortType=input  RightPortType=output  PseudoPeriodic=off  Frequencies=[]  VectorFormat=1-D array  Unit=K  AffineConversion=off
  dT_HA_d_K : nesl_utility/PS-Simulink Converter  PhysicalDomain=network_engine_domain  SubClassName=ps_output  LeftPortType=input  RightPortType=output  PseudoPeriodic=off  Frequencies=[]  VectorFormat=1-D array  Unit=K  AffineConversion=off
  i_t : Outport
  v : Outport  Port=2
  p_t : Outport  Port=3
  dT_JH_t : Outport  Port=4
  dT_HA_t : Outport  Port=5
  i_d : Outport  Port=6
  p_d : Outport  Port=7
  dT_JH_d : Outport  Port=8
  dT_HA_d : Outport  Port=9
  wires:
  i_t_A/1 -> i_t/1
  v_V/1 -> v/1
  p_t_W/1 -> p_t/1
  dT_JH_t_K/1 -> dT_JH_t/1
  dT_HA_t_K/1 -> dT_HA_t/1
  i_d_A/1 -> i_d/1
  p_d_W/1 -> p_d/1
  dT_JH_d_K/1 -> dT_JH_d/1
  dT_HA_d_K/1 -> dT_HA_d/1
  g/1 -> gate/1
  connections:
  Rth JH transistor/RConn1 -- C heatsink transistor/LConn1 -- Rth HA transistor/LConn1 -- dT JH transistor/RConn1 -- dT HA transistor/LConn1
  Rth HA transistor/RConn1 -- Tambient transistor/LConn1 -- dT HA transistor/RConn1
  dT JH transistor/RConn2 -- dT_JH_t_K/LConn1
  dT HA transistor/RConn2 -- dT_HA_t_K/LConn1
  Rth JH diode/RConn1 -- C heatsink diode/LConn1 -- Rth HA diode/LConn1 -- dT JH diode/RConn1 -- dT HA diode/LConn1
  Rth HA diode/RConn1 -- Tambient diode/LConn1 -- dT HA diode/RConn1
  dT JH diode/RConn2 -- dT_JH_d_K/LConn1
  dT HA diode/RConn2 -- dT_HA_d_K/LConn1
  gate/RConn1 -- mos_simple_2th/LConn3
  D/RConn1 -- mos_simple_2th/LConn1 -- RC snubber/LConn1 -- v_sensor/LConn1
  mos_simple_2th/RConn1 -- S/RConn1 -- RC snubber/RConn1 -- v_sensor/RConn2
  v_sensor/RConn1 -- v_V/LConn1
  mos_simple_2th/RConn3 -- p_t_W/LConn1
  mos_simple_2th/RConn4 -- p_d_W/LConn1
  mos_simple_2th/RConn5 -- i_t_A/LConn1
  mos_simple_2th/RConn6 -- i_d_A/LConn1
  mos_simple_2th/LConn2 -- Cj transistor/LConn1 -- Rth JH transistor/LConn1 -- dT JH transistor/LConn1
  mos_simple_2th/RConn2 -- Cj diode/LConn1 -- Rth JH diode/LConn1 -- dT JH diode/LConn1
